simulink model "ARDroneHoverSim_4_1"  (R2025b)
settings: Solver=ode1  StartTime=0.0  StopTime=100  FixedStep=simDT  RelTol=1e-3  EnableMultiTasking=on
values from neighbouring files (symbols this model uses):
  A = zeros(2)    [setup_4_1.m]    (also in setup_4_4.m = [0 0 -1  0)
  B = eye(2)    [setup_4_1.m]    (also in setup_4_4.m = [eye(2); zeros(2)])
  C = eye(2)    [setup_4_1.m]    (also in setup_4_4.m = [eye(2) zeros(2)])
  tStepX = 10    [setup_sim.m]
  tStepY = 30    [setup_sim.m]
  xRefStep = 1    [setup_sim.m]
  yRefStep = 1    [setup_sim.m]
undefined symbols (not defined in the file or in its folder): FMS, KALMAN_GAIN
libraries: ARBlocks x2
settings Model: Creator=Paul Freeman  LastModifiedBy=caio
settings SolverCC: AlgebraicLoopSolver=TrustRegion
settings DataIOCC: SaveFormat=Array  SignalLoggingSaveFormat=ModelDataLogs  SaveOutput=off  SignalLogging=off  ReturnWorkspaceOutputs=off
settings OptimizationCC: ExpressionDepthLimit=2147483647.0  LifeSpan=inf
settings DebuggingCC: UnderspecifiedInitializationDetection=Classic  MergeDetectMultiDrivingBlocksExec=none  SolverPrmCheckMsg=warning  MultiTaskDSMMsg=warning  MultiTaskCondExecSysMsg=none  FcnCallInpInsideContextMsg=warning  UnconnectedInputMsg=warning  UnconnectedOutputMsg=warning  UnconnectedLineMsg=warning  StateNameClashWarn=warning  SFUnexpectedBacktrackingDiag=warning  SFNoUnconditionalDefaultTransitionDiag=warning  SFExecutionAtInitializationDiag=none  ArithmeticOperatorsInVariantConditions=warning
settings HardwareCC: ProdBitPerPointer=32.0  ProdBitPerSizeT=32.0  ProdBitPerPtrDiffT=32.0  ProdLargestAtomicInteger=Long  ProdLargestAtomicFloat=Double  ProdEndianess=BigEndian  ProdWordSize=32.0  ProdHWDeviceType=Freescale->32-bit PowerPC
settings ModelReferenceCC: EnableRefExpFcnMdlSchedulingChecks=on  PropagateSignalLabelsOutOfModel=off
settings SFSimCC: SimUseLocalCustomCode=off  SimParseCustomCode=off  CustomCodeUndefinedFunction=UseInterfaceOnly
settings RTWCC: RTWUseLocalCustomCode=off  GPUComputeCapability=3.5
settings CodeAppCC: StateflowObjectComments=on
settings GRTTargetCC: TargetLangStandard=C89/C90 (ANSI)  CombineOutputUpdateFcns=off  GRTInterface=on
settings ConfigComp: CovMetricSettings=dw  CovSaveCumulativeToWorkspaceVar=on  CovSaveSingleToWorkspaceVar=on  CovExternalEMLEnable=off

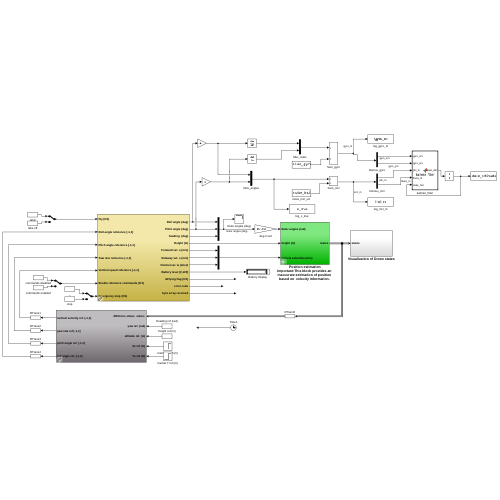
[thumbnail: Simulink's stored preview of the top-level diagram]
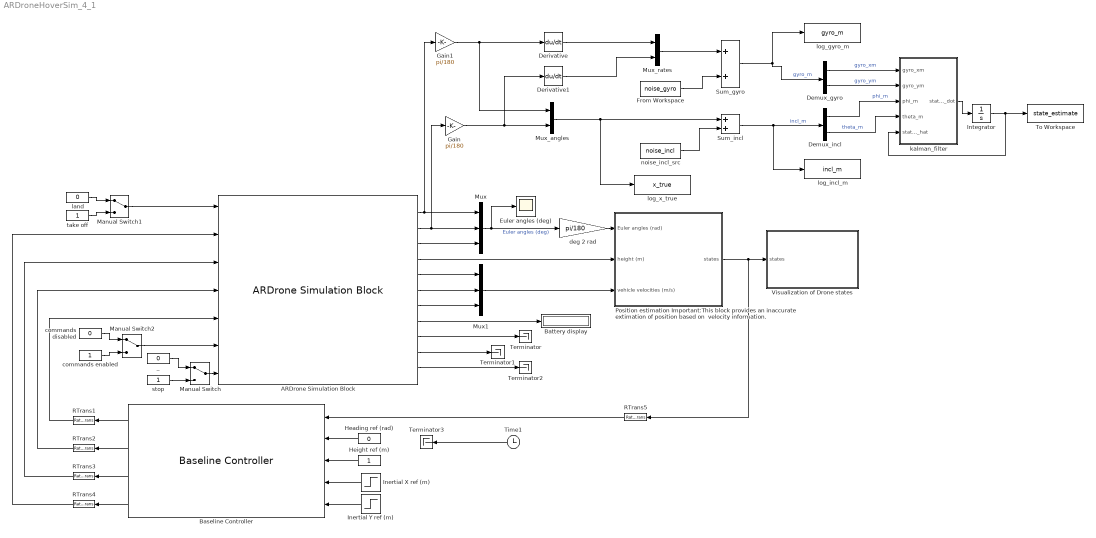
== system ARDroneHoverSim_4_1 ==
  ARDrone Simulation Block : ARBlocks/ARDrone Simulation Block  SystemSampleTime=-1  VariantActivationTime=update diagram  EmptyChoice=off  PassThrough=off  PassThroughVariantControl=(default)  EmptyChoiceVariantControl=(default)  AllowFlexibleInterface=on  Latency=0  AutoFrameSizeCalculation=off
  Baseline Controller : ARBlocks/Baseline Controller  SystemSampleTime=-1  VariantActivationTime=update diagram  EmptyChoice=off  PassThrough=off  PassThroughVariantControl=(default)  EmptyChoiceVariantControl=(default)  AllowFlexibleInterface=on  Latency=0  AutoFrameSizeCalculation=off
  Battery display : Display
  Demux_gyro : Demux  Outputs=2
  Demux_incl : Demux  Outputs=2
  Derivative : Derivative
  Derivative1 : Derivative
  Euler angles (deg) : Scope
      settings: ActiveDisplayYMinimum=-22.5  ActiveDisplayYMaximum=22.5  DataLoggingMaxPoints=500000
  From Workspace : FromWorkspace  VariableName=noise_gyro
  Gain : Gain  Gain=pi/180
  Gain1 : Gain  Gain=pi/180
  Heading ref (rad) : Constant  Value=0  SampleTime=FMS.Ts
  Height ref (m) : Constant  SampleTime=FMS.Ts
  Inertial X ref (m) : Step  Time=tStepX  After=xRefStep  SampleTime=FMS.Ts
  Inertial Y ref (m) : Step  Time=tStepY  After=yRefStep  SampleTime=FMS.Ts
  Integrator : Integrator  InitialCondition=zeros(size(A,1), 1)
  Manual Switch : ManualSwitch
  Manual Switch1 : ManualSwitch
  Manual Switch2 : ManualSwitch
  Mux : Mux  Inputs=3
  Mux1 : Mux  Inputs=3
  Mux_angles : Mux  Inputs=2
  Mux_rates : Mux  Inputs=2
  "Position estimation Important:This block provides an inaccurate extimation of position based on  velocity information. " : Subsystem  AncestorBlock=|
      | ARBlocks/Position estimation
      | Important:This block provides an 
      | inaccurate extimation of position 
      | based on  velocity information.
  RTrans{1..4} (4 alike) : RateTransition  OutPortSampleTime=simDT
  RTrans5 : RateTransition  OutPortSampleTime=FMS.Ts
  Sum_gyro : Sum
  Sum_incl : Sum
  Terminator{,1..3} (4 alike) : Terminator
  Time1 : Clock
  To Workspace : ToWorkspace  VariableName=state_estimate  SaveFormat=Structure With Time  SampleTime=-1
  Visualization of Drone states : Subsystem
  _ : Constant  Value=0
  commands disabled : Constant  Value=0
  commands enabled : Constant
  deg 2 rad : Gain  Gain=pi/180
  kalman_filter : MATLAB Function  TreatAsAtomicUnit=on
  land : Constant  Value=0
  log_gyro_m : ToWorkspace  VariableName=gyro_m  SaveFormat=Structure With Time  SampleTime=-1
  log_incl_m : ToWorkspace  VariableName=incl_m  SaveFormat=Structure With Time  SampleTime=-1
  log_x_true : ToWorkspace  VariableName=x_true  SaveFormat=Structure With Time  SampleTime=-1
  noise_incl_src : FromWorkspace  VariableName=noise_incl
  stop : Constant
  take off : Constant
  wires:
  _/1 -> Manual Switch/1
  stop/1 -> Manual Switch/2
  land/1 -> Manual Switch1/1
  take off/1 -> Manual Switch1/2
  commands disabled/1 -> Manual Switch2/1
  commands enabled/1 -> Manual Switch2/2
  Manual Switch1/1 -> ARDrone Simulation Block/1
  Manual Switch2/1 -> ARDrone Simulation Block/6
  Manual Switch/1 -> ARDrone Simulation Block/7
  ARDrone Simulation Block/5 -> Mux1/1
  ARDrone Simulation Block/6 -> Mux1/2
  ARDrone Simulation Block/7 -> Mux1/3
  Mux/1 -> Euler angles (deg)/1, deg 2 rad/1  "Euler angles (deg)"
  ARDrone Simulation Block/8 -> Battery display/1
  Baseline Controller/1 -> RTrans1/1
  Baseline Controller/3 -> RTrans3/1
  "Position estimation Important:This block provides an inaccurate extimation of position based on  velocity information. "/1(states) -> RTrans5/1, Visualization of Drone states/1(states)
  deg 2 rad/1 -> "Position estimation Important:This block provides an inaccurate extimation of position based on  velocity information. "/1(Euler angles (rad))
  ARDrone Simulation Block/4 -> "Position estimation Important:This block provides an inaccurate extimation of position based on  velocity information. "/2(height (m))
  Mux1/1 -> "Position estimation Important:This block provides an inaccurate extimation of position based on  velocity information. "/3(vehicle velocities (m/s))
  Baseline Controller/2 -> RTrans2/1
  Baseline Controller/4 -> RTrans4/1
  ARDrone Simulation Block/3 -> Mux/3
  ARDrone Simulation Block/9 -> Terminator/1
  RTrans1/1 -> ARDrone Simulation Block/5
  RTrans2/1 -> ARDrone Simulation Block/4
  RTrans3/1 -> ARDrone Simulation Block/3
  RTrans4/1 -> ARDrone Simulation Block/2
  ARDrone Simulation Block/10 -> Terminator1/1
  ARDrone Simulation Block/11 -> Terminator2/1
  Time1/1 -> Terminator3/1
  Heading ref (rad)/1 -> Baseline Controller/2
  Height ref (m)/1 -> Baseline Controller/3
  RTrans5/1 -> Baseline Controller/1
  Inertial X ref (m)/1 -> Baseline Controller/4
  Inertial Y ref (m)/1 -> Baseline Controller/5
  Integrator/1 -> kalman_filter/5(state_hat), To Workspace/1
  kalman_filter/1(state_dot) -> Integrator/1
  Demux_incl/2 -> kalman_filter/4(theta_m)  "theta_m"
  Demux_incl/1 -> kalman_filter/3(phi_m)  "phi_m"
  Demux_gyro/2 -> kalman_filter/2(gyro_ym)  "gyro_ym"
  Demux_gyro/1 -> kalman_filter/1(gyro_xm)  "gyro_xm"
  Mux_angles/1 -> Sum_incl/1, log_x_true/1
  Gain1/1 -> Mux_angles/1, Derivative/1
  Gain/1 -> Derivative1/1, Mux_angles/2
  Sum_gyro/1 -> Demux_gyro/1, log_gyro_m/1  "gyro_m"
  Sum_incl/1 -> log_incl_m/1, Demux_incl/1  "incl_m"
  Derivative/1 -> Mux_rates/1
  Derivative1/1 -> Mux_rates/2
  Mux_rates/1 -> Sum_gyro/1
  noise_incl_src/1 -> Sum_incl/2
  ARDrone Simulation Block/2 -> Mux/2, Gain/1
  ARDrone Simulation Block/1 -> Mux/1, Gain1/1
  From Workspace/1 -> Sum_gyro/2

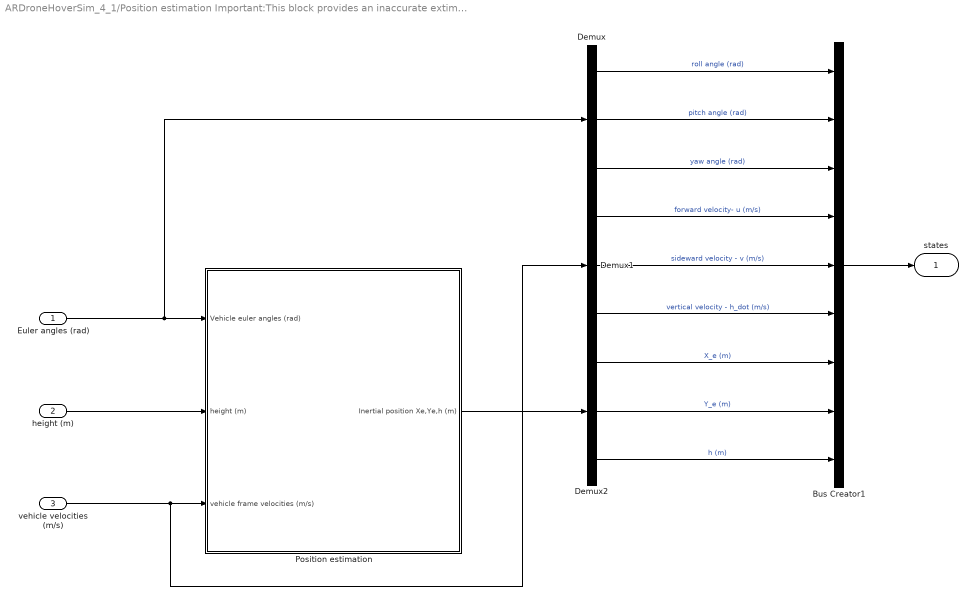
== system ARDroneHoverSim_4_1/Position estimation Important:This block provides an inaccurate extimation of position based on  velocity information.  ==
  Euler angles (rad) : Inport
  height (m) : Inport  Port=2
  vehicle velocities (m/s) : Inport  Port=3
  Bus Creator1 : BusCreator  Inputs=9
  Demux : Demux  Outputs=3
  Demux1 : Demux  Outputs=3
  Demux2 : Demux  Outputs=3
  Position estimation : Subsystem
  states : Outport
  wires:
  height (m)/1 -> Position estimation/2(height (m))
  Bus Creator1/1 -> states/1
  Demux2/3 -> Bus Creator1/9  "h (m)"
  Demux2/2 -> Bus Creator1/8  "Y_e (m)"
  Demux2/1 -> Bus Creator1/7  "X_e (m)"
  Demux1/3 -> Bus Creator1/6  "vertical velocity - h_dot (m/s)"
  Demux1/2 -> Bus Creator1/5  "sideward velocity - v (m/s)"
  Demux1/1 -> Bus Creator1/4  "forward velocity- u (m/s)"
  Demux/3 -> Bus Creator1/3  "yaw angle (rad)"
  Demux/2 -> Bus Creator1/2  "pitch angle (rad)"
  Demux/1 -> Bus Creator1/1  "roll angle (rad)"
  Position estimation/1(Inertial position Xe,Ye,h (m)) -> Demux2/1
  Euler angles (rad)/1 -> Demux/1, Position estimation/1(Vehicle euler angles (rad))
  vehicle velocities (m/s)/1 -> Position estimation/3(vehicle frame velocities (m/s)), Demux1/1

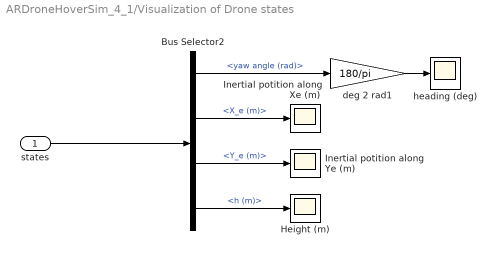
== system ARDroneHoverSim_4_1/Visualization of Drone states ==
  states : Inport
  Bus Selector2 : BusSelector  OutputSignals=yaw angle (rad),X_e (m),Y_e (m),h (m)
  Height (m) : Scope
      settings: ActiveDisplayYMinimum=-0.12689  ActiveDisplayYMaximum=1.0973  DataLoggingMaxPoints=500000  DataLoggingVariableName=ScopeData5
  Inertial potition along Xe (m) : Scope
      settings: ActiveDisplayYMinimum=-22.5  ActiveDisplayYMaximum=22.5  DataLoggingMaxPoints=500000  DataLoggingVariableName=ScopeData3
  Inertial potition along Ye (m) : Scope
      settings: ActiveDisplayYMinimum=-22.5  ActiveDisplayYMaximum=22.5  DataLoggingMaxPoints=500000  DataLoggingVariableName=ScopeData4
  deg 2 rad1 : Gain  Gain=180/pi
  heading (deg) : Scope
      settings: ActiveDisplayYMinimum=-22.5  ActiveDisplayYMaximum=22.5  DataLoggingMaxPoints=500000  DataLoggingVariableName=ScopeData2
  wires:
  states/1 -> Bus Selector2/1
  Bus Selector2/1 -> deg 2 rad1/1  "<yaw angle (rad)>"
  Bus Selector2/2 -> Inertial potition along Xe (m)/1  "<X_e (m)>"
  Bus Selector2/3 -> Inertial potition along Ye (m)/1  "<Y_e (m)>"
  Bus Selector2/4 -> Height (m)/1  "<h (m)>"
  deg 2 rad1/1 -> heading (deg)/1

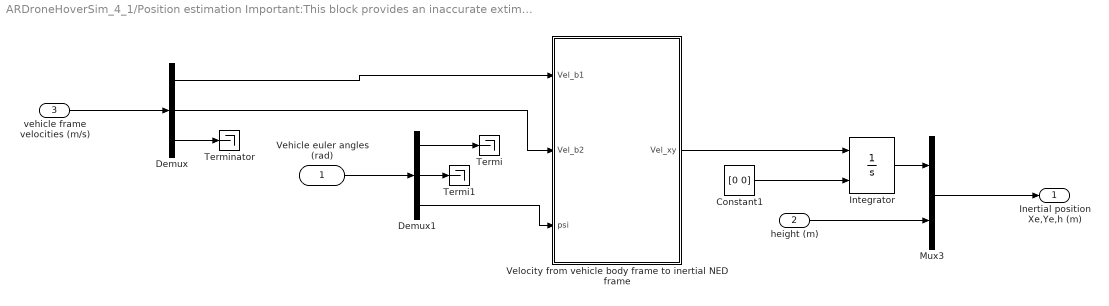
== system ARDroneHoverSim_4_1/Position estimation Important:This block provides an inaccurate extimation of position based on  velocity information. /Position estimation ==
  Vehicle euler angles (rad) : Inport
  height (m) : Inport  Port=2
  vehicle frame velocities (m/s) : Inport  Port=3
  Constant1 : Constant  Value=[0 0]
  Demux : Demux  Outputs=3
  Demux1 : Demux  Outputs=3
  Integrator : Integrator  InitialConditionSource=external
  Mux3 : Mux  Inputs=2
  Termi : Terminator
  Termi1 : Terminator
  Terminator : Terminator
  Velocity from vehicle body frame to inertial NED  frame : MATLAB Function  TreatAsAtomicUnit=on
  Inertial position Xe,Ye,h (m) : Outport
  wires:
  Mux3/1 -> Inertial position Xe,Ye,h (m)/1
  height (m)/1 -> Mux3/2
  Vehicle euler angles (rad)/1 -> Demux1/1
  vehicle frame velocities (m/s)/1 -> Demux/1
  Demux1/3 -> Velocity from vehicle body frame to inertial NED  frame/3(psi)
  Integrator/1 -> Mux3/1
  Constant1/1 -> Integrator/2
  Velocity from vehicle body frame to inertial NED  frame/1(Vel_xy) -> Integrator/1
  Demux1/2 -> Termi1/1
  Demux1/1 -> Termi/1
  Demux/1 -> Velocity from vehicle body frame to inertial NED  frame/1(Vel_b1)
  Demux/2 -> Velocity from vehicle body frame to inertial NED  frame/2(Vel_b2)
  Demux/3 -> Terminator/1

== matlab function ARDroneHoverSim_4_1/kalman_filter ==
  data: gyro_xm input; state_dot output; gyro_ym input; phi_m input; theta_m input; state_hat input; A parameter; B parameter; C parameter; KALMAN_GAIN parameter
function state_dot = kalman_filter(gyro_xm, gyro_ym, phi_m, theta_m, state_hat, A, B, C, KALMAN_GAIN)
    u = [gyro_xm; gyro_ym];     % rate gyro, rad/s
    y = [phi_m; theta_m];       % inclinometer, rad
    state_dot = A*state_hat + B*u + KALMAN_GAIN*(y - C*state_hat);
end

== matlab function ARDroneHoverSim_4_1/Position estimation Important:This block provides an inaccurate extimation of position based on  velocity information. /Position estimation/Velocity from vehicle body frame to inertial NED  frame ==
  data: Vel_b1 input; Vel_b2 input; Vel_xy output; psi input
function Vel_xy = fcn(Vel_b1, Vel_b2, psi)
%#codegen
T = [cos(psi) -sin(psi) ; sin(psi) cos(psi)] ; 
Vel_xy = T*[Vel_b1; Vel_b2];
